simulink model "radia_ltspice_pid_optuna"  (R2026a)
settings: Solver=FixedStepDiscrete  StopTime=0.80000000000000004  FixedStep=0.1
settings Model: Creator=Administrator  LastModifiedBy=Administrator

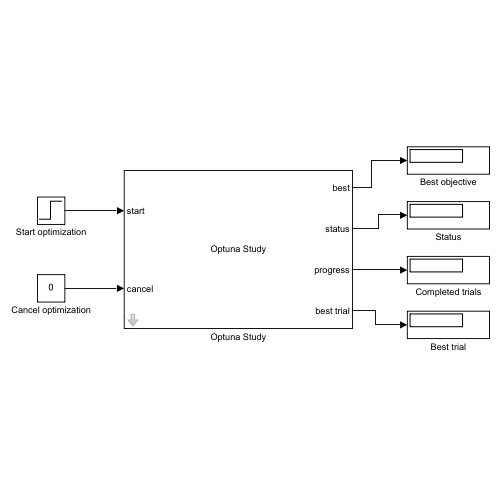
[thumbnail: Simulink's stored preview of the top-level diagram]
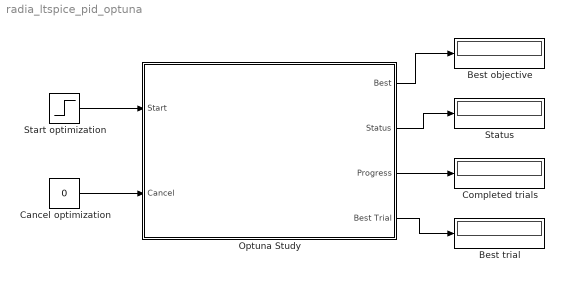
== system radia_ltspice_pid_optuna ==
  Best objective : Display
  Best trial : Display
  Cancel optimization : Constant  Value=0  SampleTime=0.1
  Completed trials : Display
  Optuna Study : Subsystem  mask{objective_fcn='radia.simulink.ltspicePIDObjective', num_trials=8, directions="minimize", storage_path='', sample_time_s=0.10000000000000001, live_visualization=off, sampler_name=cmaes, seed=[], pruner_name=none, parameter_spec=[], model_name='radia_ltspice_pid_optuna', selected_trial=-1}
      mask prompts: objective_fcn "Objective function"; num_trials "Total trial budget"; directions "Objective directions"; storage_path "Study MAT file"; sample_time_s "Trial sample time (s)"; live_visualization "External MATLAB monitor"; sampler_name "Sampler"; seed "Sampler seed ([] = fresh)"; pruner_name "Pruner"; parameter_spec "OptimizationParameter array"; model_name "Model to update"; selected_trial "Trial to apply (-1 = best)"
      mask help: Compact MATLAB-native Optuna study. Change the sampler, seed, pruner, search space, or total trial budget in this dialog and run again; the MAT study resumes without changing wiring.
      mask init:
      | set_param([gcb '/Advanced Runtime'],'Parameters','objective_fcn,num_trials,directions,storage_path,sample_time_s,strcmp(live_visualization,''on''),struct(''Name'',sampler_name,''Seed'',seed,''Pruner'',pruner_name,''Parameters'',parameter_spec,''ModelName'',model_name)');
      mask TypeOptions sampler_name: auto | random | tpe | cmaes | motpe | nsgaii | gp | nsgaiii | bruteforce | qmc
      mask TypeOptions pruner_name: none | median | hyperband | percentile | patient | successivehalving | threshold
      mask DialogControl review_study Prompt: Review saved study
      mask DialogControl review_study Callback: radia.simulink.reviewOptunaStudy(gcb);
      mask DialogControl apply_trial Prompt: Apply selected trial
      mask DialogControl apply_trial Callback: radia.simulink.applyOptunaTrial(gcb,selected_trial);
      mask Display: disp('Optuna Study');port_label('input',1,'start');port_label('input',2,'cancel');port_label('output',1,'best');port_label('output',2,'status');port_label('output',3,'progress');port_label('output',4,'best trial');
  Start optimization : Step  Time=0  SampleTime=0.1
  Status : Display
  wires:
  Start optimization/1 -> Optuna Study/1(Start)
  Optuna Study/3(Progress) -> Completed trials/1
  Cancel optimization/1 -> Optuna Study/2(Cancel)
  Optuna Study/1(Best) -> Best objective/1
  Optuna Study/2(Status) -> Status/1
  Optuna Study/4(Best Trial) -> Best trial/1

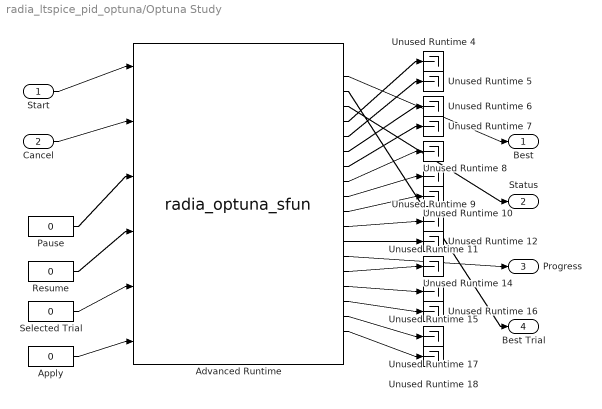
== system radia_ltspice_pid_optuna/Optuna Study ==
  Start : Inport
  Cancel : Inport  Port=2
  Advanced Runtime : M-S-Function  FunctionName=radia_optuna_sfun  Parameters=objective_fcn,num_trials,directions,storage_path,sample_time_s,strcmp(live_visualization,'on'),struct('Name',sampler_name,'Seed',seed,'Pruner',pruner_name,'Parameters',parameter_spec,'ModelName',model_name)
  Apply : Constant  Value=0
  Pause : Constant  Value=0
  Resume : Constant  Value=0
  Selected Trial : Constant  Value=0
  Unused Runtime {4..12,14..18} (14 alike) : Terminator
  Best : Outport
  Status : Outport  Port=2
  Progress : Outport  Port=3
  Best Trial : Outport  Port=4
  wires:
  Start/1 -> Advanced Runtime/1
  Cancel/1 -> Advanced Runtime/2
  Pause/1 -> Advanced Runtime/3
  Resume/1 -> Advanced Runtime/4
  Selected Trial/1 -> Advanced Runtime/5
  Apply/1 -> Advanced Runtime/6
  Advanced Runtime/1 -> Best/1
  Advanced Runtime/3 -> Status/1
  Advanced Runtime/13 -> Progress/1
  Advanced Runtime/2 -> Best Trial/1
  Advanced Runtime/4 -> Unused Runtime 4/1
  Advanced Runtime/5 -> Unused Runtime 5/1
  Advanced Runtime/6 -> Unused Runtime 6/1
  Advanced Runtime/7 -> Unused Runtime 7/1
  Advanced Runtime/8 -> Unused Runtime 8/1
  Advanced Runtime/9 -> Unused Runtime 9/1
  Advanced Runtime/10 -> Unused Runtime 10/1
  Advanced Runtime/11 -> Unused Runtime 11/1
  Advanced Runtime/12 -> Unused Runtime 12/1
  Advanced Runtime/14 -> Unused Runtime 14/1
  Advanced Runtime/15 -> Unused Runtime 15/1
  Advanced Runtime/16 -> Unused Runtime 16/1
  Advanced Runtime/17 -> Unused Runtime 17/1
  Advanced Runtime/18 -> Unused Runtime 18/1
